simulink model "Trim_model"  (R2024b)
settings: Solver=FixedStepAuto  StartTime=0.0  StopTime=10  FixedStep=0.01  RelTol=1e-3
values from neighbouring files (symbols this model uses):
  MAV = loadMAVParameters()    [computeTransferFunctions.m]
libraries: matrix_library x2
settings Model: Creator=emrec  LastModifiedBy=emrec

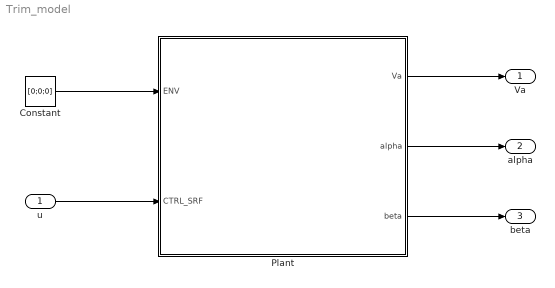
== system Trim_model ==
  u : Inport  PortDimensions=[4,1]
  Constant : Constant  Value=[0;0;0]
  Plant : Subsystem
  Va : Outport
  alpha : Outport  Port=2
  beta : Outport  Port=3
  wires:
  Constant/1 -> Plant/1(ENV)
  u/1 -> Plant/2(CTRL_SRF)
  Plant/3(beta) -> beta/1
  Plant/2(alpha) -> alpha/1
  Plant/1(Va) -> Va/1

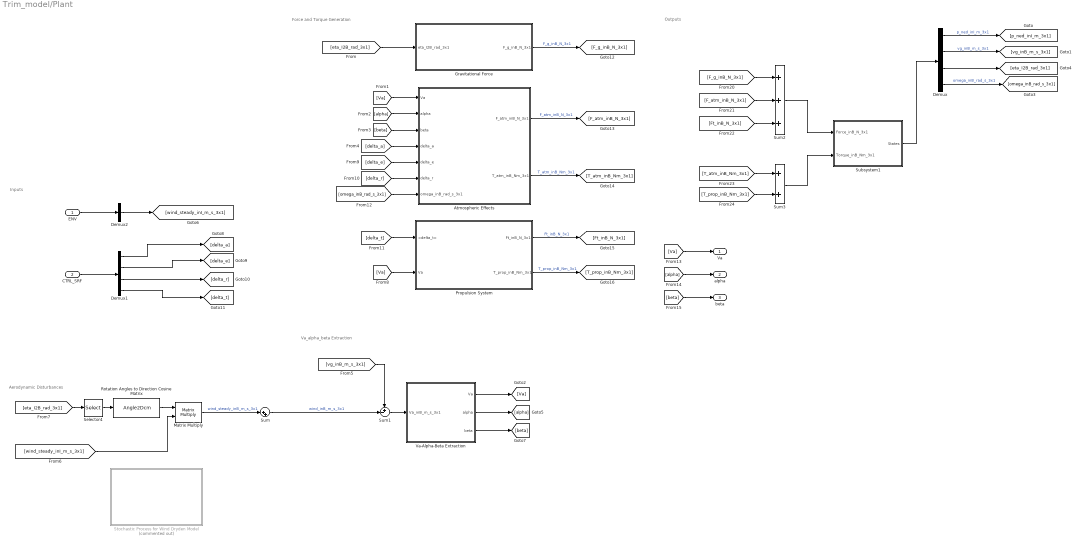
== system Trim_model/Plant ==
  note: Aerodynamic Disturbances
  note: Force and Torque Generation
  note: Inputs
  note: Outputs
  note: Va_alpha_beta Extraction
  ENV : Inport
  CTRL_SRF : Inport  Port=2
  Atmospheric Effects : Subsystem
  Demux : Demux
  Demux1 : Demux
  Demux2 : Demux  Outputs=1
  Gravitational Force : Subsystem
  Matrix Multiply : Product  Multiplication=Matrix(*)
  Propulsion System : Subsystem
  Rotation Angles to Direction Cosine Matrix : Angle2Dcm
      settings: AttributesFormatString=Rotation Order: %<rotationOrder>
  Selector4 : Selector  InputPortWidth=3  IndexOptions=Index vector (dialog)  Indices=[3 2 1]  OutputSizes=1
  Stochastic Process for Wind Dryden Model : Subsystem  Commented=on
  Subsystem1 : Subsystem  mask{init_states=MAV.init_states, J_B_B=MAV.J_B_B, m=MAV.m}
      mask prompts: init_states "Initial state values"; J_B_B "Inertia matrix (Kg.m3)"; m "Mass (Kg)"
  Sum : Sum  Inputs=|++
  Sum1 : Sum  Inputs=+-|
  Sum2 : Sum  Inputs=+++
  Sum3 : Sum
  Va-Alpha-Beta Extraction : Subsystem
  Va : Outport
  alpha : Outport  Port=2
  beta : Outport  Port=3
  wires:
  [T_prop_inB_Nm_3x1] -> Sum3/2
  [T_atm_inB_Nm_3x1] -> Sum3/1
  [Ft_inB_N_3x1] -> Sum2/3
  [F_atm_inB_N_3x1] -> Sum2/2
  [F_g_inB_N_3x1] -> Sum2/1
  Gravitational Force/1(F_g_inB_N_3x1) -> [F_g_inB_N_3x1]  "F_g_inB_N_3x1"
  Atmospheric Effects/1(F_atm_inB_N_3x1) -> [F_atm_inB_N_3x1]  "F_atm_inB_N_3x1"
  Atmospheric Effects/2(T_atm_inB_Nm_3x1) -> [T_atm_inB_Nm_3x1]  "T_atm_inB_Nm_3x1"
  Propulsion System/1(Ft_inB_N_3x1) -> [Ft_inB_N_3x1]  "Ft_inB_N_3x1"
  Propulsion System/2(T_prop_inB_Nm_3x1) -> [T_prop_inB_Nm_3x1]  "T_prop_inB_Nm_3x1"
  Demux1/2 -> [delta_e]
  ENV/1 -> Demux2/1
  Sum1/1 -> Va-Alpha-Beta Extraction/1(Va_inB_m_s_3x1)
  [wind_steady_inI_m_s_3x1] -> Matrix Multiply/2
  Demux2/1 -> [wind_steady_inI_m_s_3x1]
  [Va] -> Propulsion System/2(Va)
  Selector4/1 -> Rotation Angles to Direction Cosine Matrix/1
  Demux1/4 -> [delta_t]
  [Va] -> Atmospheric Effects/1(Va)
  Va-Alpha-Beta Extraction/1(Va) -> [Va]
  Demux/4 -> [omega_inB_rad_s_3x1]  "omega_inB_rad_s_3x1"
  [delta_r] -> Atmospheric Effects/6(delta_r)
  [delta_a] -> Atmospheric Effects/4(delta_a)
  Matrix Multiply/1 -> Sum/1  "wind_steady_inB_m_s_3x1"
  [delta_e] -> Atmospheric Effects/5(delta_e)
  Subsystem1/1(States) -> Demux/1
  [delta_t] -> Propulsion System/1(<delta_t>)
  Va-Alpha-Beta Extraction/3(beta) -> [beta]
  Demux/1 -> [p_ned_inI_m_3x1]  "p_ned_inI_m_3x1"
  CTRL_SRF/1 -> Demux1/1
  Demux1/1 -> [delta_a]
  Demux/3 -> [eta_I2B_rad_3x1]
  Sum/1 -> Sum1/2  "wind_inB_m_s_3x1"
  [vg_inB_m_s_3x1] -> Sum1/1
  Demux/2 -> [vg_inB_m_s_3x1]  "vg_inB_m_s_3x1"
  [eta_I2B_rad_3x1] -> Selector4/1
  Rotation Angles to Direction Cosine Matrix/1 -> Matrix Multiply/1
  [eta_I2B_rad_3x1] -> Gravitational Force/1(eta_I2B_rad_3x1)
  Sum3/1 -> Subsystem1/2(Torque_inB_Nm_3x1)
  Va-Alpha-Beta Extraction/2(alpha) -> [alpha]
  Sum2/1 -> Subsystem1/1(Force_inB_N_3x1)
  [alpha] -> Atmospheric Effects/2(alpha)
  [beta] -> Atmospheric Effects/3(beta)
  Demux1/3 -> [delta_r]
  [omega_inB_rad_s_3x1] -> Atmospheric Effects/7(omega_inB_rad_s_3x1)
  [beta] -> beta/1
  [Va] -> Va/1
  [alpha] -> alpha/1

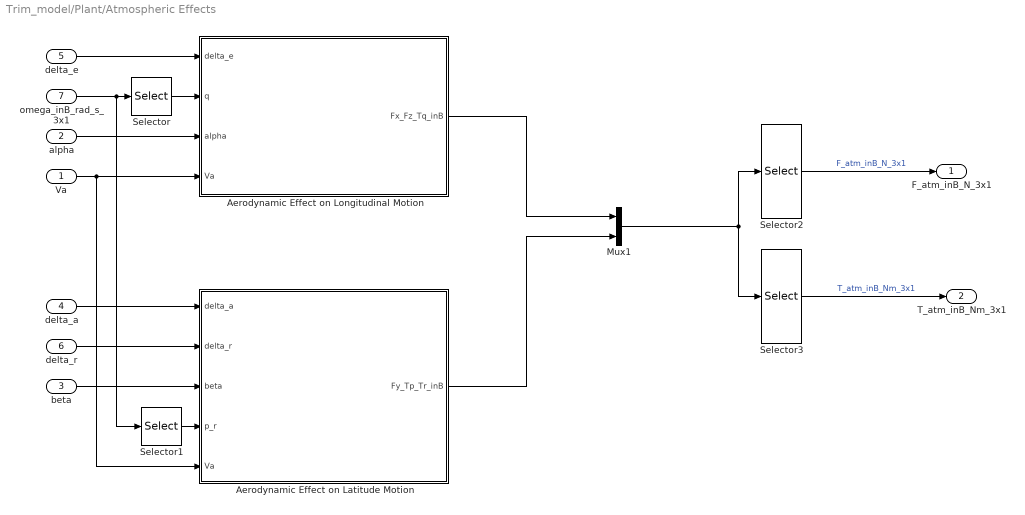
== system Trim_model/Plant/Atmospheric Effects ==
  Va : Inport
  alpha : Inport  Port=2
  beta : Inport  Port=3
  delta_a : Inport  Port=4
  delta_e : Inport  Port=5
  delta_r : Inport  Port=6
  omega_inB_rad_s_3x1 : Inport  Port=7
  Aerodynamic Effect on Latitude Motion : Subsystem
  Aerodynamic Effect on Longitudinal Motion : Subsystem
  Mux1 : Mux  Inputs=2
  Selector : Selector  InputPortWidth=3  IndexOptions=Index vector (dialog)  Indices=[2]  OutputSizes=1
  Selector1 : Selector  InputPortWidth=3  IndexOptions=Index vector (dialog)  Indices=[1 3]  OutputSizes=1
  Selector2 : Selector  InputPortWidth=6  IndexOptions=Index vector (dialog)  Indices=[1 4 2]  OutputSizes=1
  Selector3 : Selector  InputPortWidth=6  IndexOptions=Index vector (dialog)  Indices=[5 3 6]  OutputSizes=1
  F_atm_inB_N_3x1 : Outport
  T_atm_inB_Nm_3x1 : Outport  Port=2
  wires:
  Mux1/1 -> Selector3/1, Selector2/1
  Selector2/1 -> F_atm_inB_N_3x1/1  "F_atm_inB_N_3x1"
  delta_e/1 -> Aerodynamic Effect on Longitudinal Motion/1(delta_e)
  delta_a/1 -> Aerodynamic Effect on Latitude Motion/1(delta_a)
  Aerodynamic Effect on Longitudinal Motion/1(Fx_Fz_Tq_inB) -> Mux1/1
  alpha/1 -> Aerodynamic Effect on Longitudinal Motion/3(alpha)
  Aerodynamic Effect on Latitude Motion/1(Fy_Tp_Tr_inB) -> Mux1/2
  delta_r/1 -> Aerodynamic Effect on Latitude Motion/2(delta_r)
  omega_inB_rad_s_3x1/1 -> Selector1/1, Selector/1
  Va/1 -> Aerodynamic Effect on Latitude Motion/5(Va), Aerodynamic Effect on Longitudinal Motion/4(Va)
  beta/1 -> Aerodynamic Effect on Latitude Motion/3(beta)
  Selector3/1 -> T_atm_inB_Nm_3x1/1  "T_atm_inB_Nm_3x1"
  Selector/1 -> Aerodynamic Effect on Longitudinal Motion/2(q)
  Selector1/1 -> Aerodynamic Effect on Latitude Motion/4(p_r)

== system Trim_model/Plant/Gravitational Force ==
  eta_I2B_rad_3x1 : Inport
  Constant : Constant  Value=MAV.m * MAV.g
  Product : Product
  R_B_I_c3 : MATLAB Function  TreatAsAtomicUnit=on
  F_g_inB_N_3x1 : Outport
  wires:
  eta_I2B_rad_3x1/1 -> R_B_I_c3/1(u)
  R_B_I_c3/1(y) -> Product/1
  Constant/1 -> Product/2  "F_g_inI_N_3x1"
  Product/1 -> F_g_inB_N_3x1/1  "F_g_inB_N_3x1"

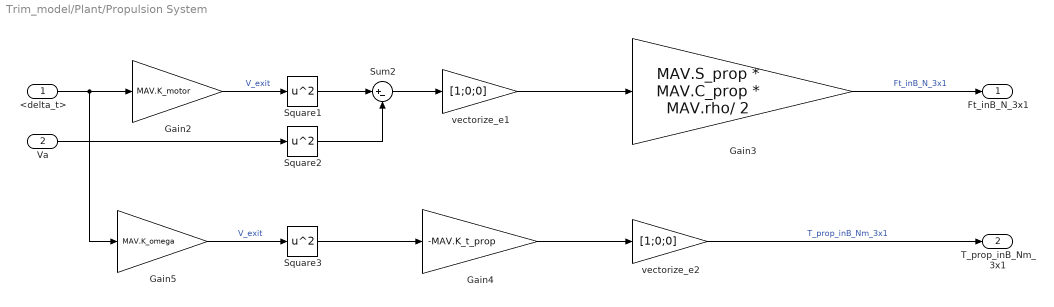
== system Trim_model/Plant/Propulsion System ==
  <delta_t> : Inport
  Va : Inport  Port=2
  Gain2 : Gain  Gain=MAV.K_motor
  Gain3 : Gain  Gain=MAV.S_prop * MAV.C_prop * MAV.rho/ 2
  Gain4 : Gain  Gain=-MAV.K_t_prop
  Gain5 : Gain  Gain=MAV.K_omega
  Square1 : Math  Operator=square
  Square2 : Math  Operator=square
  Square3 : Math  Operator=square
  Sum2 : Sum  Inputs=|+-
  vectorize_e1 : Gain  Gain=[1;0;0]
  vectorize_e2 : Gain  Gain=[1;0;0]
  Ft_inB_N_3x1 : Outport
  T_prop_inB_Nm_3x1 : Outport  Port=2
  wires:
  Gain2/1 -> Square1/1  "V_exit"
  Square1/1 -> Sum2/1
  Gain4/1 -> vectorize_e2/1
  Sum2/1 -> vectorize_e1/1
  Square2/1 -> Sum2/2
  vectorize_e1/1 -> Gain3/1
  Gain3/1 -> Ft_inB_N_3x1/1  "Ft_inB_N_3x1"
  <delta_t>/1 -> Gain2/1, Gain5/1
  Va/1 -> Square2/1
  vectorize_e2/1 -> T_prop_inB_Nm_3x1/1  "T_prop_inB_Nm_3x1"
  Square3/1 -> Gain4/1
  Gain5/1 -> Square3/1  "V_exit"

== system Trim_model/Plant/Stochastic Process for Wind Dryden Model ==

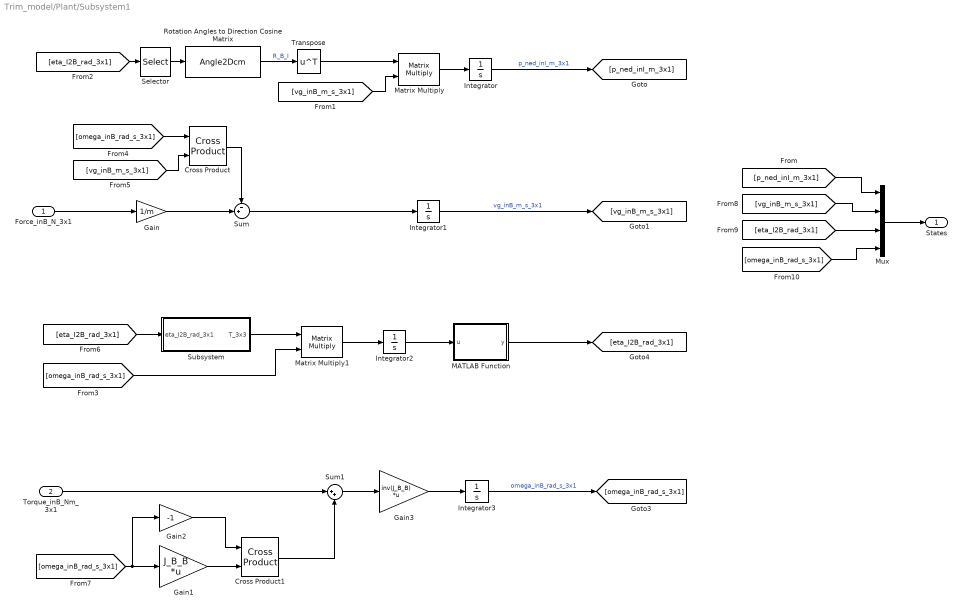
== system Trim_model/Plant/Subsystem1 ==
  Force_inB_N_3x1 : Inport
  Torque_inB_Nm_3x1 : Inport  Port=2
  Cross Product : matrix_library/Cross Product
  Cross Product1 : matrix_library/Cross Product
  Gain : Gain  Gain=1/m
  Gain1 : Gain  Gain=J_B_B  Multiplication=Matrix(K*u)
  Gain2 : Gain  Gain=-1
  Gain3 : Gain  Gain=inv(J_B_B)  Multiplication=Matrix(K*u)
  Integrator : Integrator  InitialCondition=init_states(1:3)
  Integrator1 : Integrator  InitialCondition=init_states(4:6)
  Integrator2 : Integrator  InitialCondition=init_states(7:9)
  Integrator3 : Integrator  InitialCondition=init_states(10:12)
  MATLAB Function : MATLAB Function  TreatAsAtomicUnit=on
  Matrix Multiply : Product  Multiplication=Matrix(*)
  Matrix Multiply1 : Product  Multiplication=Matrix(*)
  Mux : Mux
  Rotation Angles to Direction Cosine Matrix : Angle2Dcm
      settings: AttributesFormatString=Rotation Order: %<rotationOrder>
  Selector : Selector  InputPortWidth=3  IndexOptions=Index vector (dialog)  Indices=[3;2;1]  OutputSizes=1
  Subsystem : Subsystem
  Sum : Sum  Inputs=-+|
  Sum1 : Sum  Inputs=|++
  Transpose : Math  Operator=transpose
  States : Outport
  wires:
  Gain3/1 -> Integrator3/1
  [p_ned_inI_m_3x1] -> Mux/1
  [omega_inB_rad_s_3x1] -> Cross Product/1
  Matrix Multiply1/1 -> Integrator2/1
  Gain1/1 -> Cross Product1/2
  [eta_I2B_rad_3x1] -> Subsystem/1(eta_I2B_rad_3x1)
  [omega_inB_rad_s_3x1] -> Matrix Multiply1/2
  Integrator1/1 -> [vg_inB_m_s_3x1]  "vg_inB_m_s_3x1"
  [vg_inB_m_s_3x1] -> Cross Product/2
  Selector/1 -> Rotation Angles to Direction Cosine Matrix/1
  [eta_I2B_rad_3x1] -> Selector/1
  Cross Product/1 -> Sum/1
  Integrator/1 -> [p_ned_inI_m_3x1]  "p_ned_inI_m_3x1"
  Matrix Multiply/1 -> Integrator/1
  Force_inB_N_3x1/1 -> Gain/1
  Rotation Angles to Direction Cosine Matrix/1 -> Transpose/1  "R_B_I"
  [omega_inB_rad_s_3x1] -> Gain2/1, Gain1/1
  Mux/1 -> States/1
  [omega_inB_rad_s_3x1] -> Mux/4
  Transpose/1 -> Matrix Multiply/1
  Integrator3/1 -> [omega_inB_rad_s_3x1]  "omega_inB_rad_s_3x1"
  [vg_inB_m_s_3x1] -> Matrix Multiply/2
  [eta_I2B_rad_3x1] -> Mux/3
  Torque_inB_Nm_3x1/1 -> Sum1/1
  Gain2/1 -> Cross Product1/1
  Sum1/1 -> Gain3/1
  Integrator2/1 -> MATLAB Function/1(u)
  [vg_inB_m_s_3x1] -> Mux/2
  Subsystem/1(T_3x3) -> Matrix Multiply1/1
  Cross Product1/1 -> Sum1/2
  Sum/1 -> Integrator1/1
  Gain/1 -> Sum/2
  MATLAB Function/1(y) -> [eta_I2B_rad_3x1]

== system Trim_model/Plant/Va-Alpha-Beta Extraction ==
  note: Va >= ||vr|| -> Va = 0 -> vr = 0
  note: Switch is removed to test whether it causes
      | the trim error.
  Va_inB_m_s_3x1 : Inport
  Asin : Trigonometry  Operator=asin
  Constant : Constant  Value=1e-4
  Demux : Demux  Outputs=3
  Divide1 : Product  Inputs=*/
  Saturation : Saturate  UpperLimit=1  LowerLimit=-1
  Sum : Sum  Inputs=|++
  Trigonometric Function : Trigonometry  Operator=atan2  OutputSignalType=real
  norm2 : Subsystem
  Va : Outport
  alpha : Outport  Port=2
  beta : Outport  Port=3
  wires:
  Va_inB_m_s_3x1/1 -> Demux/1, norm2/1(Va_inB_m_s_3x1)
  Asin/1 -> beta/1
  Demux/1 -> Trigonometric Function/2  "ur"
  Demux/2 -> Divide1/1  "vr"
  Trigonometric Function/1 -> alpha/1
  Sum/1 -> Divide1/2
  Saturation/1 -> Asin/1
  Divide1/1 -> Saturation/1
  Constant/1 -> Sum/2
  norm2/1(Va) -> Sum/1, Va/1  "Va"
  Demux/3 -> Trigonometric Function/1  "wr"

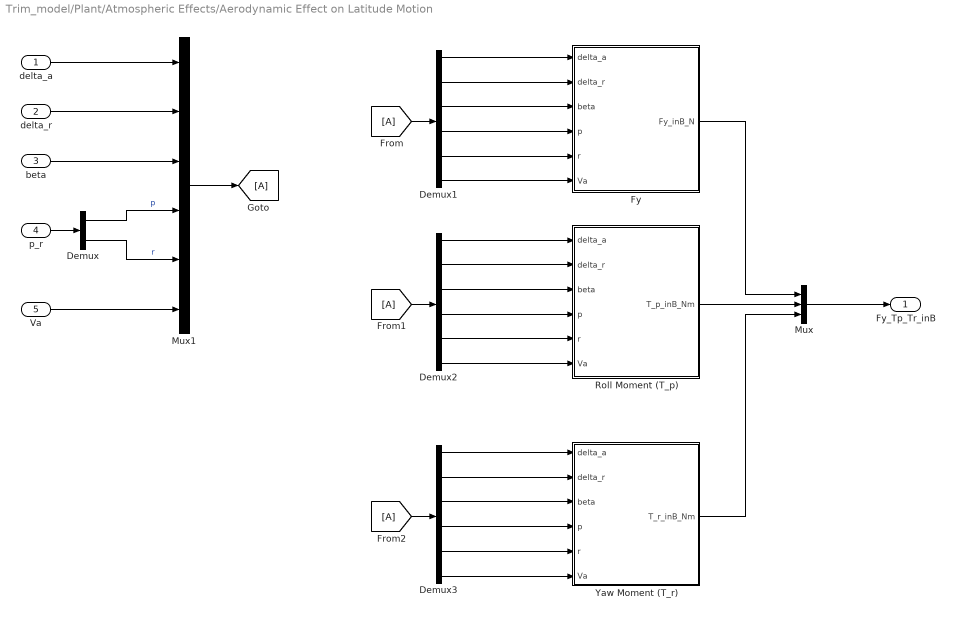
== system Trim_model/Plant/Atmospheric Effects/Aerodynamic Effect on Latitude Motion ==
  delta_a : Inport
  delta_r : Inport  Port=2
  beta : Inport  Port=3
  p_r : Inport  Port=4
  Va : Inport  Port=5
  Demux : Demux  Outputs=2
  Demux1 : Demux  Outputs=6
  Demux2 : Demux  Outputs=6
  Demux3 : Demux  Outputs=6
  From : From
  From1 : From
  From2 : From
  Fy : Subsystem
  Goto : Goto
  Mux : Mux  Inputs=3
  Mux1 : Mux  Inputs=6
  Roll Moment (T_p) : Subsystem
  Yaw Moment (T_r) : Subsystem
  Fy_Tp_Tr_inB : Outport
  wires:
  Mux/1 -> Fy_Tp_Tr_inB/1
  p_r/1 -> Demux/1
  Fy/1(Fy_inB_N) -> Mux/1
  Roll Moment (T_p)/1(T_p_inB_Nm) -> Mux/2
  Yaw Moment (T_r)/1(T_r_inB_Nm) -> Mux/3
  Demux1/1 -> Fy/1(delta_a)
  delta_a/1 -> Mux1/1
  delta_r/1 -> Mux1/2
  beta/1 -> Mux1/3
  Demux/1 -> Mux1/4  "p"
  Demux/2 -> Mux1/5  "r"
  Va/1 -> Mux1/6
  Mux1/1 -> Goto/1
  From/1 -> Demux1/1
  Demux1/2 -> Fy/2(delta_r)
  Demux1/3 -> Fy/3(beta)
  Demux1/4 -> Fy/4(p)
  Demux1/5 -> Fy/5(r)
  Demux1/6 -> Fy/6(Va)
  Demux2/4 -> Roll Moment (T_p)/4(p)
  Demux2/5 -> Roll Moment (T_p)/5(r)
  From1/1 -> Demux2/1
  Demux2/2 -> Roll Moment (T_p)/2(delta_r)
  Demux2/1 -> Roll Moment (T_p)/1(delta_a)
  Demux2/6 -> Roll Moment (T_p)/6(Va)
  Demux2/3 -> Roll Moment (T_p)/3(beta)
  Demux3/4 -> Yaw Moment (T_r)/4(p)
  Demux3/5 -> Yaw Moment (T_r)/5(r)
  From2/1 -> Demux3/1
  Demux3/2 -> Yaw Moment (T_r)/2(delta_r)
  Demux3/1 -> Yaw Moment (T_r)/1(delta_a)
  Demux3/6 -> Yaw Moment (T_r)/6(Va)
  Demux3/3 -> Yaw Moment (T_r)/3(beta)

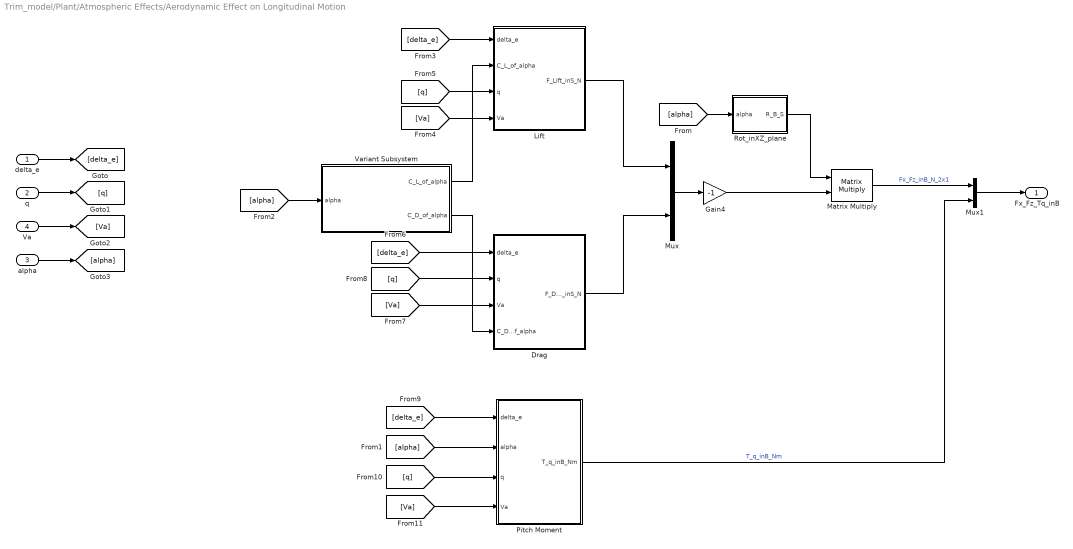
== system Trim_model/Plant/Atmospheric Effects/Aerodynamic Effect on Longitudinal Motion ==
  delta_e : Inport
  q : Inport  Port=2
  alpha : Inport  Port=3
  Va : Inport  Port=4
  Drag : Subsystem
  Gain4 : Gain  Gain=-1
  "Lift " : Subsystem
  Matrix Multiply : Product  Multiplication=Matrix(*)
  Mux : Mux  Inputs=2
  Mux1 : Mux  Inputs=2
  Pitch Moment : Subsystem
  Rot_inXZ_plane : MATLAB Function  TreatAsAtomicUnit=on
  Variant Subsystem : Subsystem  Variant=on
  Fx_Fz_Tq_inB : Outport
  wires:
  alpha/1 -> [alpha]
  [alpha] -> Rot_inXZ_plane/1(alpha)
  Mux/1 -> Gain4/1
  Rot_inXZ_plane/1(R_B_S) -> Matrix Multiply/1
  Gain4/1 -> Matrix Multiply/2
  Matrix Multiply/1 -> Mux1/1  "Fx_Fz_inB_N_2x1"
  Variant Subsystem/1(C_L_of_alpha) -> "Lift "/2(C_L_of_alpha)
  "Lift "/1(F_Lift_inS_N) -> Mux/1
  Variant Subsystem/2(C_D_of_alpha) -> Drag/4(C_D_of_alpha)
  Drag/1(F_Drag_inS_N) -> Mux/2
  Pitch Moment/1(T_q_inB_Nm) -> Mux1/2  "T_q_inB_Nm"
  Mux1/1 -> Fx_Fz_Tq_inB/1
  delta_e/1 -> [delta_e]
  Va/1 -> [Va]
  q/1 -> [q]
  [alpha] -> Variant Subsystem/1(alpha)
  [delta_e] -> "Lift "/1(delta_e)
  [Va] -> "Lift "/4(Va)
  [q] -> "Lift "/3(q)
  [delta_e] -> Drag/1(delta_e)
  [q] -> Drag/2(q)
  [Va] -> Drag/3(Va)
  [delta_e] -> Pitch Moment/1(delta_e)
  [q] -> Pitch Moment/3(q)
  [Va] -> Pitch Moment/4(Va)
  [alpha] -> Pitch Moment/2(alpha)

== system Trim_model/Plant/Subsystem1/Subsystem ==
  eta_I2B_rad_3x1 : Inport
  MATLAB Function : MATLAB Function  TreatAsAtomicUnit=on
  T_3x3 : Outport
  wires:
  eta_I2B_rad_3x1/1 -> MATLAB Function/1(u)
  MATLAB Function/1(y) -> T_3x3/1

== system Trim_model/Plant/Va-Alpha-Beta Extraction/norm2 ==
  Va_inB_m_s_3x1 : Inport
  Sqrt : Sqrt
  Square : Math  Operator=square
  Sum of Elements : Sum  Inputs=+
  Va : Outport
  wires:
  Sqrt/1 -> Va/1
  Sum of Elements/1 -> Sqrt/1
  Square/1 -> Sum of Elements/1
  Va_inB_m_s_3x1/1 -> Square/1

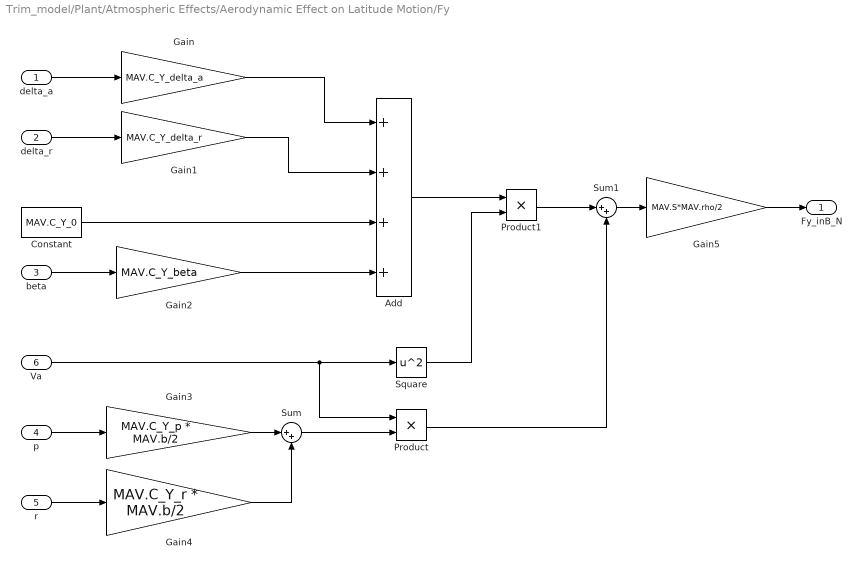
== system Trim_model/Plant/Atmospheric Effects/Aerodynamic Effect on Latitude Motion/Fy ==
  delta_a : Inport
  delta_r : Inport  Port=2
  beta : Inport  Port=3
  p : Inport  Port=4
  r : Inport  Port=5
  Va : Inport  Port=6
  Add : Sum  Inputs=++++
  Constant : Constant  Value=MAV.C_Y_0
  Gain : Gain  Gain=MAV.C_Y_delta_a
  Gain1 : Gain  Gain=MAV.C_Y_delta_r
  Gain2 : Gain  Gain=MAV.C_Y_beta
  Gain3 : Gain  Gain=MAV.C_Y_p * MAV.b/2
  Gain4 : Gain  Gain=MAV.C_Y_r * MAV.b/2
  Gain5 : Gain  Gain=MAV.S*MAV.rho/2
  Product : Product
  Product1 : Product
  Square : Math  Operator=square
  Sum : Sum  Inputs=|++
  Sum1 : Sum  Inputs=|++
  Fy_inB_N : Outport
  wires:
  delta_a/1 -> Gain/1
  delta_r/1 -> Gain1/1
  Constant/1 -> Add/3
  beta/1 -> Gain2/1
  Gain2/1 -> Add/4
  p/1 -> Gain3/1
  r/1 -> Gain4/1
  Gain3/1 -> Sum/1
  Gain4/1 -> Sum/2
  Gain/1 -> Add/1
  Gain1/1 -> Add/2
  Sum/1 -> Product/2
  Va/1 -> Square/1, Product/1
  Add/1 -> Product1/1
  Square/1 -> Product1/2
  Product1/1 -> Sum1/1
  Product/1 -> Sum1/2
  Sum1/1 -> Gain5/1
  Gain5/1 -> Fy_inB_N/1

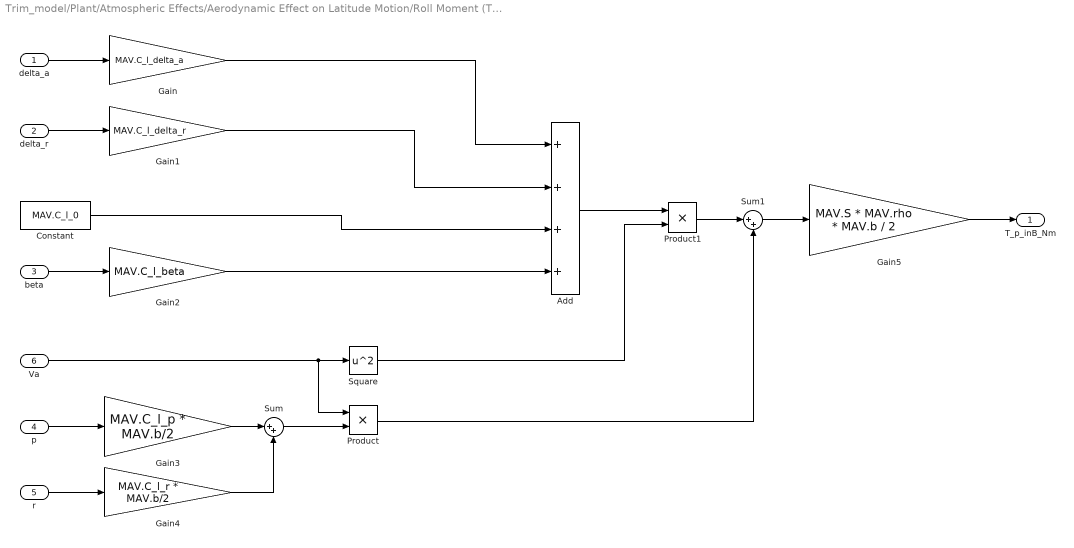
== system Trim_model/Plant/Atmospheric Effects/Aerodynamic Effect on Latitude Motion/Roll Moment (T_p) ==
  delta_a : Inport
  delta_r : Inport  Port=2
  beta : Inport  Port=3
  p : Inport  Port=4
  r : Inport  Port=5
  Va : Inport  Port=6
  Add : Sum  Inputs=++++
  Constant : Constant  Value=MAV.C_l_0
  Gain : Gain  Gain=MAV.C_l_delta_a
  Gain1 : Gain  Gain=MAV.C_l_delta_r
  Gain2 : Gain  Gain=MAV.C_l_beta
  Gain3 : Gain  Gain=MAV.C_l_p * MAV.b/2
  Gain4 : Gain  Gain=MAV.C_l_r * MAV.b/2
  Gain5 : Gain  Gain=MAV.S * MAV.rho * MAV.b / 2
  Product : Product
  Product1 : Product
  Square : Math  Operator=square
  Sum : Sum  Inputs=|++
  Sum1 : Sum  Inputs=|++
  T_p_inB_Nm : Outport
  wires:
  Gain1/1 -> Add/2
  Gain/1 -> Add/1
  Va/1 -> Square/1, Product/1
  Sum/1 -> Product/2
  Gain4/1 -> Sum/2
  Gain3/1 -> Sum/1
  r/1 -> Gain4/1
  p/1 -> Gain3/1
  Gain2/1 -> Add/4
  beta/1 -> Gain2/1
  Constant/1 -> Add/3
  delta_r/1 -> Gain1/1
  delta_a/1 -> Gain/1
  Add/1 -> Product1/1
  Square/1 -> Product1/2
  Product1/1 -> Sum1/1
  Product/1 -> Sum1/2
  Sum1/1 -> Gain5/1
  Gain5/1 -> T_p_inB_Nm/1

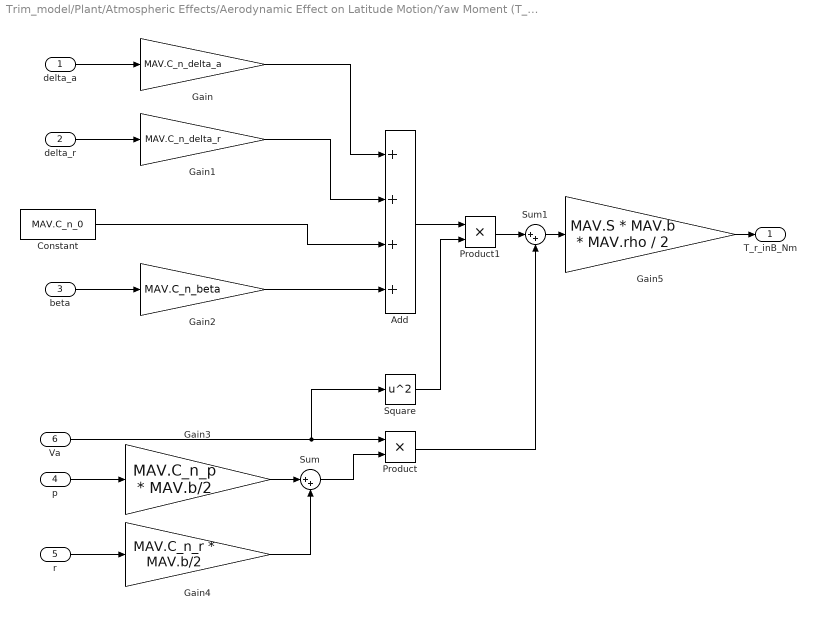
== system Trim_model/Plant/Atmospheric Effects/Aerodynamic Effect on Latitude Motion/Yaw Moment (T_r) ==
  delta_a : Inport
  delta_r : Inport  Port=2
  beta : Inport  Port=3
  p : Inport  Port=4
  r : Inport  Port=5
  Va : Inport  Port=6
  Add : Sum  Inputs=++++
  Constant : Constant  Value=MAV.C_n_0
  Gain : Gain  Gain=MAV.C_n_delta_a
  Gain1 : Gain  Gain=MAV.C_n_delta_r
  Gain2 : Gain  Gain=MAV.C_n_beta
  Gain3 : Gain  Gain=MAV.C_n_p * MAV.b/2
  Gain4 : Gain  Gain=MAV.C_n_r * MAV.b/2
  Gain5 : Gain  Gain=MAV.S * MAV.b * MAV.rho / 2
  Product : Product
  Product1 : Product
  Square : Math  Operator=square
  Sum : Sum  Inputs=|++
  Sum1 : Sum  Inputs=|++
  T_r_inB_Nm : Outport
  wires:
  Gain2/1 -> Add/4
  Constant/1 -> Add/3
  Gain1/1 -> Add/2
  delta_a/1 -> Gain/1
  p/1 -> Gain3/1
  Sum/1 -> Product/2
  Gain/1 -> Add/1
  r/1 -> Gain4/1
  Va/1 -> Square/1, Product/1
  Gain3/1 -> Sum/1
  delta_r/1 -> Gain1/1
  beta/1 -> Gain2/1
  Gain4/1 -> Sum/2
  Add/1 -> Product1/1
  Square/1 -> Product1/2
  Product1/1 -> Sum1/1
  Product/1 -> Sum1/2
  Sum1/1 -> Gain5/1
  Gain5/1 -> T_r_inB_Nm/1

== system Trim_model/Plant/Atmospheric Effects/Aerodynamic Effect on Longitudinal Motion/Drag ==
  delta_e : Inport
  q : Inport  Port=2
  Va : Inport  Port=3
  C_D_of_alpha : Inport  Port=4
  Gain : Gain  Gain=MAV.S * MAV.rho / 2
  Gain2 : Gain  Gain=MAV.C_D_delta_e
  Gain3 : Gain  Gain=MAV.C_D_q * MAV.c / 2
  Product : Product
  Product1 : Product
  Square : Math  Operator=square
  Sum : Sum  Inputs=|++
  Sum1 : Sum  Inputs=|++
  F_Drag_inS_N : Outport
  wires:
  Gain2/1 -> Sum/2
  delta_e/1 -> Gain2/1
  C_D_of_alpha/1 -> Sum/1
  q/1 -> Gain3/1
  Va/1 -> Square/1, Product/1
  Gain3/1 -> Product/2
  Sum/1 -> Product1/1
  Square/1 -> Product1/2
  Product1/1 -> Sum1/1
  Product/1 -> Sum1/2
  Sum1/1 -> Gain/1
  Gain/1 -> F_Drag_inS_N/1

== system Trim_model/Plant/Atmospheric Effects/Aerodynamic Effect on Longitudinal Motion/Lift  ==
  delta_e : Inport
  C_L_of_alpha : Inport  Port=2
  q : Inport  Port=3
  Va : Inport  Port=4
  Gain : Gain  Gain=MAV.C_L_delta_e
  Gain1 : Gain  Gain=MAV.C_L_q * MAV.c / 2
  Gain2 : Gain  Gain=MAV.S * MAV.rho / 2
  Product : Product
  Product1 : Product
  Square : Math  Operator=square
  Sum : Sum  Inputs=|++
  Sum1 : Sum  Inputs=|++
  F_Lift_inS_N : Outport
  wires:
  Gain/1 -> Sum/1
  C_L_of_alpha/1 -> Sum/2
  delta_e/1 -> Gain/1
  q/1 -> Gain1/1
  Gain1/1 -> Product/2
  Va/1 -> Product/1, Square/1
  Sum/1 -> Product1/1
  Square/1 -> Product1/2
  Product1/1 -> Sum1/1
  Product/1 -> Sum1/2
  Sum1/1 -> Gain2/1
  Gain2/1 -> F_Lift_inS_N/1

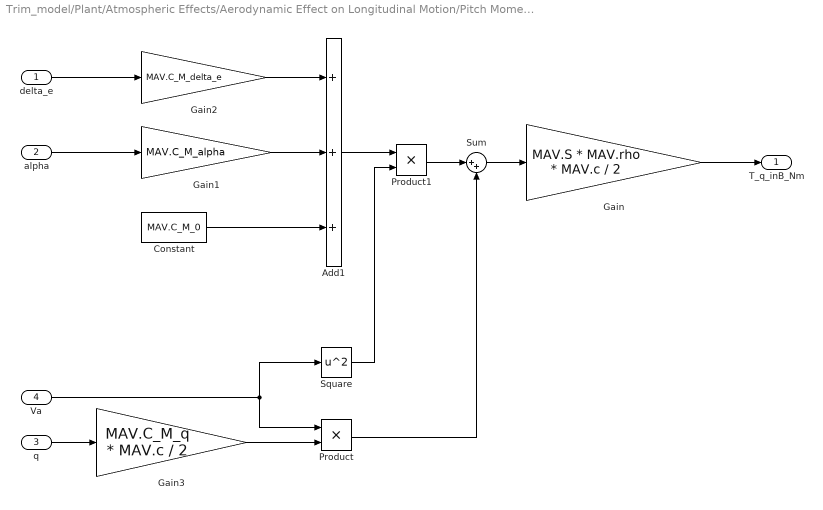
== system Trim_model/Plant/Atmospheric Effects/Aerodynamic Effect on Longitudinal Motion/Pitch Moment ==
  delta_e : Inport
  alpha : Inport  Port=2
  q : Inport  Port=3
  Va : Inport  Port=4
  Add1 : Sum  Inputs=+++
  Constant : Constant  Value=MAV.C_M_0
  Gain : Gain  Gain=MAV.S * MAV.rho * MAV.c / 2
  Gain1 : Gain  Gain=MAV.C_M_alpha
  Gain2 : Gain  Gain=MAV.C_M_delta_e
  Gain3 : Gain  Gain=MAV.C_M_q * MAV.c / 2
  Product : Product
  Product1 : Product
  Square : Math  Operator=square
  Sum : Sum  Inputs=|++
  T_q_inB_Nm : Outport
  wires:
  delta_e/1 -> Gain2/1
  Gain2/1 -> Add1/1
  alpha/1 -> Gain1/1
  Gain1/1 -> Add1/2
  Constant/1 -> Add1/3
  q/1 -> Gain3/1
  Gain3/1 -> Product/2
  Va/1 -> Product/1, Square/1
  Add1/1 -> Product1/1
  Square/1 -> Product1/2
  Product1/1 -> Sum/1
  Product/1 -> Sum/2
  Sum/1 -> Gain/1
  Gain/1 -> T_q_inB_Nm/1

== system Trim_model/Plant/Atmospheric Effects/Aerodynamic Effect on Longitudinal Motion/Variant Subsystem ==
  note: 1) Add Subsystem or Model blocks as valid variant choices.
      | 2) You cannot connect blocks at this level. At simulation, connectivity is automatically
      | determined, based on the active variant and port name matching.
  alpha : Inport
  Linear Lift Drag Effect of Alpha : Subsystem  VariantControl=LNG_MODEL == 1
  Nonlinear Lift Drag Effect of Alpha : Subsystem  VariantControl=LNG_MODEL == 2
  C_L_of_alpha : Outport
  C_D_of_alpha : Outport  Port=2

== system Trim_model/Plant/Atmospheric Effects/Aerodynamic Effect on Longitudinal Motion/Variant Subsystem/Linear Lift Drag Effect of Alpha ==
  alpha : Inport
  Constant : Constant  Value=MAV.C_L0_
  Constant1 : Constant  Value=MAV.C_D0_
  Gain : Gain  Gain=MAV.C_L_alpha
  Gain1 : Gain  Gain=MAV.C_D_alpha
  Sum : Sum  Inputs=++|
  Sum1 : Sum  Inputs=|++
  C_L_of_alpha : Outport
  C_D_of_alpha : Outport  Port=2
  wires:
  Gain/1 -> Sum/2
  Constant/1 -> Sum/1
  Sum/1 -> C_L_of_alpha/1
  alpha/1 -> Gain1/1, Gain/1
  Gain1/1 -> Sum1/1
  Constant1/1 -> Sum1/2
  Sum1/1 -> C_D_of_alpha/1

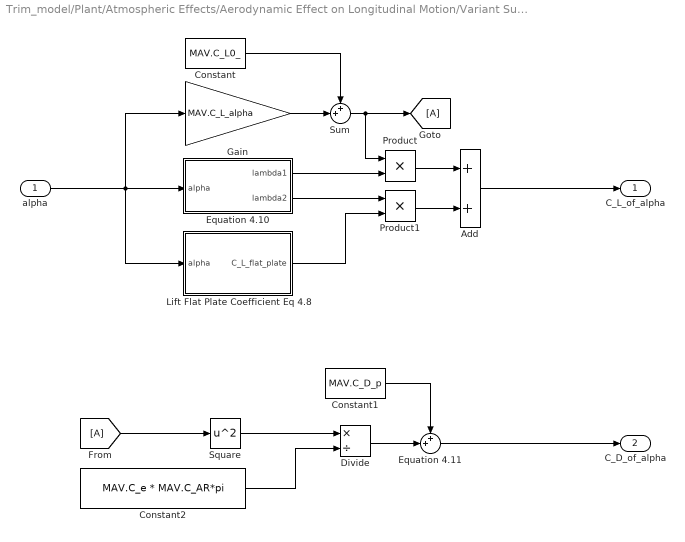
== system Trim_model/Plant/Atmospheric Effects/Aerodynamic Effect on Longitudinal Motion/Variant Subsystem/Nonlinear Lift Drag Effect of Alpha ==
  alpha : Inport
  Add : Sum
  Constant : Constant  Value=MAV.C_L0_
  Constant1 : Constant  Value=MAV.C_D_p
  Constant2 : Constant  Value=MAV.C_e * MAV.C_AR*pi
  Divide : Product  Inputs=*/
  Equation 4.10 : MATLAB Function  TreatAsAtomicUnit=on
  Equation 4.11 : Sum  Inputs=++|
  From : From
  Gain : Gain  Gain=MAV.C_L_alpha
  Goto : Goto
  Lift Flat Plate Coefficient Eq 4.8 : Subsystem
  Product : Product
  Product1 : Product
  Square : Math  Operator=square
  Sum : Sum  Inputs=++|
  C_L_of_alpha : Outport
  C_D_of_alpha : Outport  Port=2
  wires:
  Constant/1 -> Sum/1
  alpha/1 -> Lift Flat Plate Coefficient Eq 4.8/1(alpha), Equation 4.10/1(alpha), Gain/1
  Gain/1 -> Sum/2
  Sum/1 -> Goto/1, Product/1
  Equation 4.10/1(lambda1) -> Product/2
  Equation 4.10/2(lambda2) -> Product1/1
  Lift Flat Plate Coefficient Eq 4.8/1(C_L_flat_plate) -> Product1/2
  Product/1 -> Add/1
  Product1/1 -> Add/2
  Add/1 -> C_L_of_alpha/1
  From/1 -> Square/1
  Square/1 -> Divide/1
  Constant2/1 -> Divide/2
  Divide/1 -> Equation 4.11/2
  Constant1/1 -> Equation 4.11/1
  Equation 4.11/1 -> C_D_of_alpha/1

== system Trim_model/Plant/Atmospheric Effects/Aerodynamic Effect on Longitudinal Motion/Variant Subsystem/Nonlinear Lift Drag Effect of Alpha/Lift Flat Plate Coefficient Eq 4.8 ==
  alpha : Inport
  Cos : Trigonometry  Operator=cos
  Gain : Gain  Gain=2
  Product : Product  Inputs=3
  Sign : Signum
  Sin : Trigonometry
  Square : Math  Operator=square
  C_L_flat_plate : Outport
  wires:
  alpha/1 -> Cos/1, Sin/1, Sign/1
  Sin/1 -> Square/1
  Product/1 -> Gain/1
  Cos/1 -> Product/3
  Square/1 -> Product/2
  Sign/1 -> Product/1
  Gain/1 -> C_L_flat_plate/1

== matlab function Trim_model/Plant/Atmospheric Effects/Aerodynamic Effect on Longitudinal Motion/Rot_inXZ_plane ==
  data: alpha input; R_B_S output
function R_B_S = fcn(alpha)
    R_B_S = [-sin(alpha) cos(alpha);
             cos(alpha) sin(alpha)];
end

== matlab function Trim_model/Plant/Atmospheric Effects/Aerodynamic Effect on Longitudinal Motion/Variant Subsystem/Nonlinear Lift Drag Effect of Alpha/Equation 4.10 ==
  data: alpha input; lambda1 output; MAV parameter; lambda2 output
function [lambda1, lambda2] = fcn(alpha, MAV)
% Equation 4.9 - 4.10    
exp_m = exp(-MAV.M * (alpha - MAV.alpha_0));
exp_p = exp(MAV.M * (alpha + MAV.alpha_0));
lambda2 = ( 1 + exp_m + exp_p) / ((1 + exp_m)*(1 + exp_p));
lambda1 = 1 - lambda2;
end

== matlab function Trim_model/Plant/Gravitational Force/R_B_I_c3 ==
  data: u input; y output
function y = fcn(u)
    y = zeros(3,1);
    y(1) = -sin(u(2));
    y(2) = cos(u(2)) * sin(u(1));
    y(3) = cos(u(2)) * cos(u(1));
end

== matlab function Trim_model/Plant/Subsystem1/Subsystem/MATLAB Function ==
  data: u input; y output
function y = fcn(u)
    sphi = sin(u(1));
    cphi = cos(u(1));

    sthe = sin(u(2));
    cthe = cos(u(2));

    scthe = 1 / cthe;
    tthe = scthe * sthe;

    y = [1 sphi * tthe cphi*tthe;
         0 cphi -sphi;
         0 sphi*scthe cphi*scthe];

== matlab function Trim_model/Plant/Subsystem1/MATLAB Function ==
  data: u input; y output
function y = fcn(u)
    y = wrapToPi(u);
end
